simulink model "Single_Phase_Inverter"  (R2021a)
settings: Solver=VariableStepAuto  StartTime=0.0  StopTime=10.0  RelTol=1e-3
undefined symbols (not defined in the file): m
libraries: spsDCVoltageSourceLib x1, spsMultimeterLib x1, simulink x1, spsSeriesRLCBranchLib x1, spsVoltageMeasurementLib x1, spspowerguiLib x1
settings Model: Creator=45276  LastModifiedBy=45276
settings DebuggingCC: UnconnectedInputMsg=none  UnconnectedOutputMsg=none  UnconnectedLineMsg=none

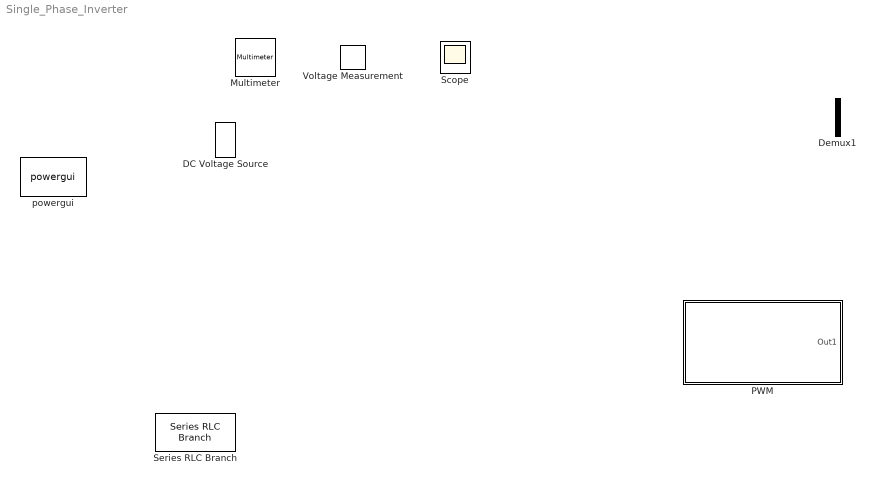
== system Single_Phase_Inverter ==
  DC Voltage Source : spsDCVoltageSourceLib/DC Voltage Source  Amplitude=100  Measurements=None
  Demux1 : Demux  Outputs=1  BusSelectionMode=on
  Multimeter : spsMultimeterLib/Multimeter  PhasorSimulation=off  OutputType=Complex  sel=1  L=1  Gain=1  yselected={}  PSBOutputType=1  PSBequivalent=0  AxesSetting=[0,0.1,-100,100]  Display=0  SavedBlockNames=-11
  PWM : Subsystem  mask{m=m, fc=750}
      mask prompts: m "m(0<m<=1)"; fc "fc(Hz)"
      mask TypeOptions m: Constant/Value
      mask TypeOptions fc:
      | Repeating
      | Sequence/rep_seq_t
  Scope : Scope
  Series RLC Branch : spsSeriesRLCBranchLib/Series RLC Branch  LConnTagsString=__new0  RConnTagsString=__new0  BranchType=RL  Resistance=1  Inductance=2e-3  SetiL0=off  InitialCurrent=0  Capacitance=1e-6  Setx0=off  InitialVoltage=0  Measurements=None
  Voltage Measurement : spsVoltageMeasurementLib/Voltage Measurement  PhasorSimulation=off  OutputType=Complex  PSBequivalent=0
  powergui : spspowerguiLib/powergui  Priority=1  SimulationMode=Discrete  SampleTime=1e-5  frequency=60  Iterations=50  frequencyindice=0  Pbase=100e6  ErrMax=1e-4  UnitsV=kV  UnitsW=MW  buscounter=0  FunctionMessages=off  echomessages=off  EnableUseOfTLC=off  CurrentSourceSwitches=off  DisableSnubberDevices=off  DisableRonSwitches=off  DisableVfSwitches=off  DisplayEquations=off  AutomaticDiscreteSolvers=off  SolverType=Tustin/Backward Euler (TBE)  Interpol=off  ExternalGateDelay=off  methode=off  Ts=100  x0status=blocks  SPID=off  SwTol=0  HookPort=off  NonlinearTolerance=1e-4  nMaxIteration=100  ContinueOnMaxIteration=off  RestoreLinks=warning  ResistiveCurrentMeasurement=off  Frange=[0:2:500]  Ylog=off  Xlog=on  ShowGrid=off  save=off  variable=ZData  structure=0  ZoomFFT=off  StartTime=0.0  cycles=1  DisplayStyle=1  fundamental=60  FreqAxis=off  MaxFrequency=1000  frequencyindicesteady=1  RmsSteady=1  display=off

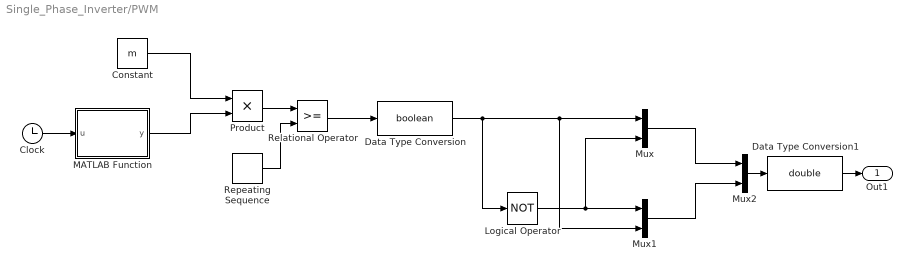
== system Single_Phase_Inverter/PWM ==
  Clock : Clock
  Constant : Constant  Value=m
  Data Type Conversion : DataTypeConversion  OutDataTypeStr=boolean
  Data Type Conversion1 : DataTypeConversion  OutDataTypeStr=double
  Logical Operator : Logic  Operator=NOT  AllPortsSameDT=off  OutDataTypeStr=boolean
  MATLAB Function : MATLAB Function  TreatAsAtomicUnit=on
  Mux : Mux  Inputs=2
  Mux1 : Mux  Inputs=2
  Mux2 : Mux  Inputs=2
  Product : Product
  Relational Operator : RelationalOperator  OutDataTypeStr=boolean  RndMeth=Simplest
  Repeating Sequence : simulink/Sources/Repeating Sequence  rep_seq_t=fc  rep_seq_y=[0-1 1 0]
  Out1 : Outport
  wires:
  Logical Operator/1 -> Mux/2, Mux1/1
  Relational Operator/1 -> Data Type Conversion/1
  Product/1 -> Relational Operator/1
  Repeating Sequence/1 -> Relational Operator/2
  Mux2/1 -> Data Type Conversion1/1
  Data Type Conversion/1 -> Mux1/2, Mux/1, Logical Operator/1
  Mux/1 -> Mux2/1
  Clock/1 -> MATLAB Function/1(u)
  MATLAB Function/1(y) -> Product/2
  Mux1/1 -> Mux2/2
  Constant/1 -> Product/1
  Data Type Conversion1/1 -> Out1/1

== matlab function Single_Phase_Inverter/PWM/MATLAB Function ==
  data: u input; y output
function y = fcn(u)

    y = sin(2*pi*f*u);
end
